simulink model "ups_final"  (R2026b)
settings: Solver=VariableStepAuto  StopTime=0.1
libraries: simulink x1
settings Model: Creator=Arnav  LastModifiedBy=Arnav

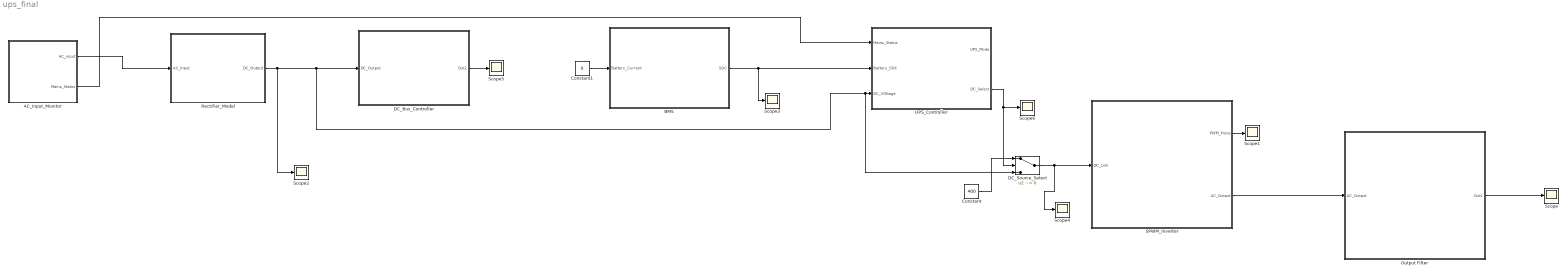
== system ups_final ==
  AC_Input_Monitor : Subsystem
  BMS : Subsystem
  Constant : Constant  Value=400
  Constant1 : Constant  Value=0
  DC_Bus_Controller : Subsystem
  DC_Source_Select : Switch  Criteria=u2 ~= 0  SaturateOnIntegerOverflow=off  InputSameDT=off
  Output FIlter : Subsystem
  Rectifier_Model : Subsystem
  SPWM_Inverter : Subsystem
  Scope{,1..6} (7 alike) : Scope
      Scope settings: ActiveDisplayYMinimum=-381.20518861891435  ActiveDisplayYMaximum=378.57896074089928
      Scope1 settings: ActiveDisplayYMinimum=-1.1322580645161295  ActiveDisplayYMaximum=1.072741935483871
      Scope2 settings: ActiveDisplayYMinimum=-46.016919146523243  ActiveDisplayYMaximum=94.97510292967813  DataLoggingVariableName=ScopeData2
      Scope3 settings: ActiveDisplayYMinimum=40  ActiveDisplayYMaximum=60  DataLoggingVariableName=ScopeData3
      Scope4 settings: ActiveDisplayYMinimum=-245.56913487976578  ActiveDisplayYMaximum=689.39592911034924  DataLoggingVariableName=ScopeData4
      Scope5 settings: ActiveDisplayYMinimum=395.31020492389047  ActiveDisplayYMaximum=442.20815568498574  DataLoggingVariableName=ScopeData5
      Scope6 settings: ActiveDisplayYMinimum=0.642662889893993  ActiveDisplayYMaximum=1.4502887347945048  DataLoggingVariableName=ScopeData6
  UPS_Controller : Subsystem
  wires:
  AC_Input_Monitor/1(AC_input) -> Rectifier_Model/1(AC_Input)
  Rectifier_Model/1(DC_Output) -> Scope2/1, DC_Bus_Controller/1(DC_Output), DC_Source_Select/3, UPS_Controller/3(DC_VOltage)
  BMS/1(SOC) -> Scope3/1, UPS_Controller/2(Battery_SOC)
  DC_Source_Select/1 -> Scope4/1, SPWM_Inverter/1(DC_Link)
  SPWM_Inverter/2(AC_Output) -> Output FIlter/1(AC_Output)
  Output FIlter/1(Out1) -> Scope/1
  SPWM_Inverter/1(PWM_Pulse) -> Scope1/1
  UPS_Controller/2(DC_Select) -> Scope6/1, DC_Source_Select/2
  DC_Bus_Controller/1(Out1) -> Scope5/1
  Constant1/1 -> BMS/1(Battery_Current)
  Constant/1 -> DC_Source_Select/1
  AC_Input_Monitor/2(Mains_Status) -> UPS_Controller/1(Mains_Status)

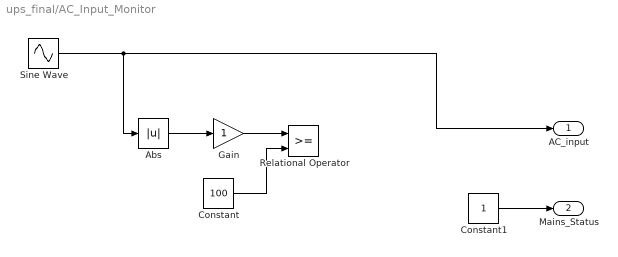
== system ups_final/AC_Input_Monitor ==
  Abs : Abs  SaturateOnIntegerOverflow=off
  Constant : Constant  Value=100
  Constant1 : Constant
  Gain : Gain
  Relational Operator : RelationalOperator  OutDataTypeStr=boolean  RndMeth=Simplest  InputSameDT=off
  Sine Wave : Sin  Amplitude=325  Frequency=2*pi*50  SampleTime=0
  AC_input : Outport
  Mains_Status : Outport  Port=2
  wires:
  Sine Wave/1 -> Abs/1, AC_input/1
  Abs/1 -> Gain/1
  Gain/1 -> Relational Operator/1
  Constant/1 -> Relational Operator/2
  Constant1/1 -> Mains_Status/1

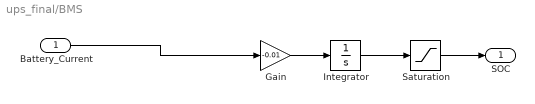
== system ups_final/BMS ==
  Battery_Current : Inport
  Gain : Gain  Gain=-0.01
  Integrator : Integrator  InitialCondition=50
  Saturation : Saturate  UpperLimit=100  LowerLimit=0
  SOC : Outport
  wires:
  Integrator/1 -> Saturation/1
  Battery_Current/1 -> Gain/1
  Gain/1 -> Integrator/1
  Saturation/1 -> SOC/1

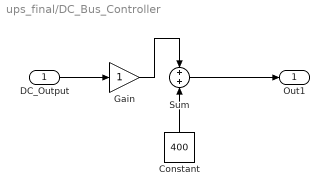
== system ups_final/DC_Bus_Controller ==
  DC_Output : Inport
  Constant : Constant  Value=400
  Gain : Gain
  Sum : Sum
  Out1 : Outport
  wires:
  DC_Output/1 -> Gain/1
  Gain/1 -> Sum/1
  Constant/1 -> Sum/2
  Sum/1 -> Out1/1

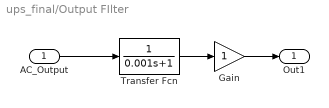
== system ups_final/Output FIlter ==
  AC_Output : Inport
  Gain : Gain
  Transfer Fcn : TransferFcn  Denominator=[0.001 1]
  Out1 : Outport
  wires:
  AC_Output/1 -> Transfer Fcn/1
  Transfer Fcn/1 -> Gain/1
  Gain/1 -> Out1/1

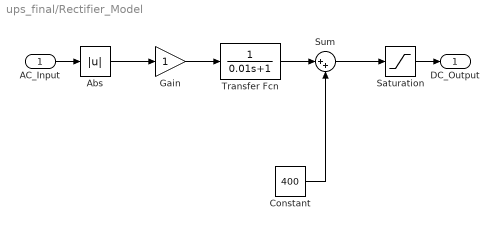
== system ups_final/Rectifier_Model ==
  AC_Input : Inport
  Abs : Abs  SaturateOnIntegerOverflow=off
  Constant : Constant  Value=400
  Gain : Gain
  Saturation : Saturate  UpperLimit=400  LowerLimit=0
  Sum : Sum  Inputs=|++
  Transfer Fcn : TransferFcn  Denominator=[0.01 1]
  DC_Output : Outport
  wires:
  AC_Input/1 -> Abs/1
  Abs/1 -> Gain/1
  Gain/1 -> Transfer Fcn/1
  Transfer Fcn/1 -> Sum/1
  Constant/1 -> Sum/2
  Saturation/1 -> DC_Output/1
  Sum/1 -> Saturation/1

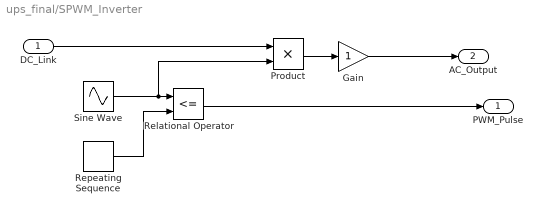
== system ups_final/SPWM_Inverter ==
  DC_Link : Inport
  Gain : Gain
  Product : Product
  Relational Operator : RelationalOperator  Operator=<=  OutDataTypeStr=boolean  RndMeth=Simplest  InputSameDT=off
  Repeating Sequence : simulink/Sources/Repeating Sequence  rep_seq_t=[0 0.00025 0.0005]  rep_seq_y=[-1 1 -1]
  Sine Wave : Sin  Amplitude=0.8  Frequency=2*pi*50  SampleTime=0
  PWM_Pulse : Outport
  AC_Output : Outport  Port=2
  wires:
  Sine Wave/1 -> Product/2, Relational Operator/1
  Repeating Sequence/1 -> Relational Operator/2
  Relational Operator/1 -> PWM_Pulse/1
  DC_Link/1 -> Product/1
  Product/1 -> Gain/1
  Gain/1 -> AC_Output/1

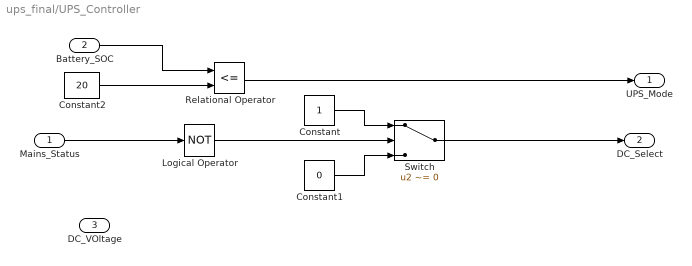
== system ups_final/UPS_Controller ==
  Mains_Status : Inport
  Battery_SOC : Inport  Port=2
  DC_VOltage : Inport  Port=3
  Constant : Constant
  Constant1 : Constant  Value=0
  Constant2 : Constant  Value=20
  Logical Operator : Logic  Operator=NOT  AllPortsSameDT=off  OutDataTypeStr=boolean
  Relational Operator : RelationalOperator  Operator=<=  OutDataTypeStr=boolean  RndMeth=Simplest  InputSameDT=off
  Switch : Switch  Criteria=u2 ~= 0  SaturateOnIntegerOverflow=off  InputSameDT=off
  UPS_Mode : Outport
  DC_Select : Outport  Port=2
  wires:
  Battery_SOC/1 -> Relational Operator/1
  Constant2/1 -> Relational Operator/2
  Mains_Status/1 -> Logical Operator/1
  Logical Operator/1 -> Switch/2
  Constant/1 -> Switch/1
  Constant1/1 -> Switch/3
  Switch/1 -> DC_Select/1
  Relational Operator/1 -> UPS_Mode/1
